simulink model "CruiseControl_V1"  (R2021b)
settings: Solver=FixedStepAuto  StartTime=0.0  StopTime=30  FixedStep=Ts  RelTol=1e-3
undefined symbols (not defined in the file): A, Cd, Crr, DiscIntNeverNeededParam, FaultInjection, FbrakeMax, Fmax, g, Kaw, ki, kp, Mass, rho, Ts, V0
settings Model: SimulationMode=software-in-the-loop (sil)  SILPILSimulationModeModelRef=accelerator  Creator=QNH2KOR  LastModifiedBy=QNH2KOR
settings OptimizationCC: DefaultParameterBehavior=Inlined  EnhancedBackFolding=on  PassReuseOutputArgsAs=Individual arguments  ZeroExternalMemoryAtStartup=off  ZeroInternalMemoryAtStartup=off  OptimizeBlockOrder=speed  DifferentSizesBufferReuse=on  OptimizationCustomize=off  EfficientTunableParamExpr=on
settings DebuggingCC: ParameterTunabilityLossMsg=error
settings SFSimCC: MATLABDynamicMemAlloc=off
settings RTWCC: Description=Embedded Coder  SystemTargetFile=ert.tlc  GenCodeOnly=on  TemplateMakefile=ert_default_tmf
settings CodeAppCC: ForceParamTrailComments=on  IgnoreCustomStorageClasses=off  OperatorAnnotations=on  SimulinkDataObjDesc=on  SFDataObjDesc=on  InsertBlockDesc=on
settings ERTTargetCC: TargetLangStandard=C99 (ISO)  GenerateSampleERTMain=on  SupportContinuousTime=on  InlinedParameterPlacement=NonHierarchical  ERTCustomFileTemplate=example_file_process.tlc

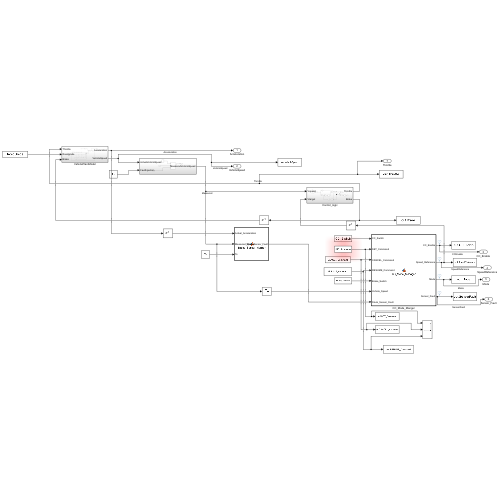
[thumbnail: Simulink's stored preview of the top-level diagram]
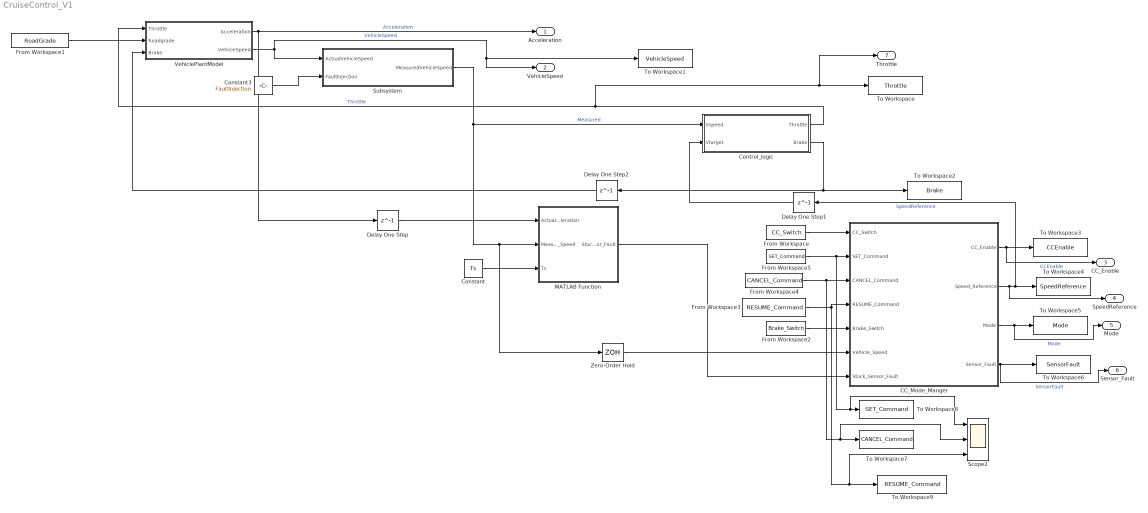
== system CruiseControl_V1 ==
  CC_Mode_Manger : MATLAB Function  TreatAsAtomicUnit=on
  Constant : Constant  Value=Ts
  Constant3 : Constant  Value=FaultInjection  SampleTime=Ts
  Control_logic : Subsystem
  Delay One Step : Delay  DelayLength=1  SampleTime=Ts
  Delay One Step1 : Delay  DelayLength=1  SampleTime=Ts
  Delay One Step2 : Delay  DelayLength=1  SampleTime=Ts
  From Workspace : FromWorkspace  VariableName=CC_Switch  SampleTime=Ts
  From Workspace1 : FromWorkspace  VariableName=RoadGrade  SampleTime=Ts  Interpolate=off  OutputAfterFinalValue=Holding final value
  From Workspace2 : FromWorkspace  VariableName=Brake_Switch  SampleTime=Ts
  From Workspace3 : FromWorkspace  VariableName=RESUME_Command  SampleTime=-1  Interpolate=off  OutputAfterFinalValue=Setting to zero
  From Workspace4 : FromWorkspace  VariableName=CANCEL_Command  SampleTime=Ts  Interpolate=off  OutputAfterFinalValue=Setting to zero
  From Workspace5 : FromWorkspace  VariableName=SET_Command  SampleTime=Ts  Interpolate=off  OutputAfterFinalValue=Setting to zero
  MATLAB Function : MATLAB Function  TreatAsAtomicUnit=on
  Scope2 : Scope  NumInputPorts=3
  Subsystem : Subsystem
  To Workspace : ToWorkspace  VariableName=Throttle  SaveFormat=Timeseries  SampleTime=-1
  To Workspace1 : ToWorkspace  VariableName=VehicleSpeed  SaveFormat=Timeseries  SampleTime=-1
  To Workspace2 : ToWorkspace  VariableName=Brake  SaveFormat=Timeseries  SampleTime=-1
  To Workspace3 : ToWorkspace  VariableName=CCEnable  SaveFormat=Timeseries  SampleTime=-1
  To Workspace4 : ToWorkspace  VariableName=SpeedReference  SaveFormat=Timeseries  SampleTime=-1
  To Workspace5 : ToWorkspace  VariableName=Mode  SaveFormat=Timeseries  SampleTime=-1
  To Workspace6 : ToWorkspace  VariableName=SensorFault  SaveFormat=Timeseries  SampleTime=-1
  To Workspace7 : ToWorkspace  VariableName=CANCEL_Command  SaveFormat=Timeseries  SampleTime=-1
  To Workspace8 : ToWorkspace  VariableName=SET_Command  SaveFormat=Timeseries  SampleTime=-1
  To Workspace9 : ToWorkspace  VariableName=RESUME_Command  SaveFormat=Timeseries  SampleTime=-1
  VehiclePlantModel : Subsystem
  Zero-Order Hold : ZeroOrderHold  SampleTime=-1
  Acceleration : Outport
  VehicleSpeed : Outport  Port=2
  CC_Enable : Outport  Port=3
  SpeedReference : Outport  Port=4
  Mode : Outport  Port=5
  Sensor_Fault : Outport  Port=6
  Throttle : Outport  Port=7
  wires:
  Control_logic/1(Throttle) -> Throttle/1, To Workspace/1, VehiclePlantModel/1(Throttle)  "Throttle"
  From Workspace1/1 -> VehiclePlantModel/2(Roadgrade)
  VehiclePlantModel/1(Acceleration) -> Acceleration/1, Delay One Step/1  "Acceleration"
  CC_Mode_Manger/1(CC_Enable) -> CC_Enable/1, To Workspace3/1  "CCEnable"
  Control_logic/2(Brake) -> Delay One Step2/1, To Workspace2/1
  VehiclePlantModel/2(VehicleSpeed) -> Subsystem/1(ActualVehicleSpeed), VehicleSpeed/1, To Workspace1/1  "VehicleSpeed"
  Constant3/1 -> Subsystem/2(FaultInjection)
  Constant/1 -> MATLAB Function/3(Ts)
  MATLAB Function/1(Stuck_Sensor_Fault) -> CC_Mode_Manger/7(Stuck_Sensor_Fault)
  From Workspace/1 -> CC_Mode_Manger/1(CC_Switch)
  From Workspace5/1 -> Scope2/1, To Workspace8/1, CC_Mode_Manger/2(SET_Command)
  From Workspace4/1 -> Scope2/2, To Workspace7/1, CC_Mode_Manger/3(CANCEL_Command)
  From Workspace3/1 -> CC_Mode_Manger/4(RESUME_Command), Scope2/3, To Workspace9/1
  From Workspace2/1 -> CC_Mode_Manger/5(Brake_Switch)
  CC_Mode_Manger/3(Mode) -> Mode/1, To Workspace5/1  "Mode"
  CC_Mode_Manger/2(Speed_Reference) -> SpeedReference/1, Delay One Step1/1, To Workspace4/1  "SpeedReference"
  Subsystem/1(MeasuredVehicleSpeed) -> Zero-Order Hold/1, MATLAB Function/2(Measured_Speed), Control_logic/1(Vspeed)  "Measured"
  Delay One Step/1 -> MATLAB Function/1(Actual_Acceleration)
  Delay One Step2/1 -> VehiclePlantModel/3(Brake)
  Delay One Step1/1 -> Control_logic/2(Vtarget)
  Zero-Order Hold/1 -> CC_Mode_Manger/6(Vehicle_Speed)
  CC_Mode_Manger/4(Sensor_Fault) -> Sensor_Fault/1, To Workspace6/1  "SensorFault"

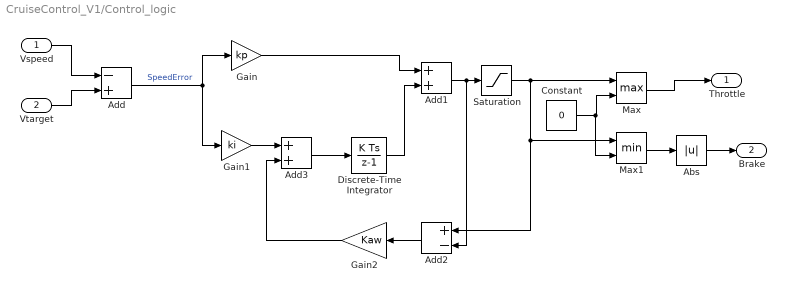
== system CruiseControl_V1/Control_logic ==
  Vspeed : Inport
  Vtarget : Inport  Port=2
  Abs : Abs
  Add : Sum  Inputs=-+
  Add1 : Sum
  Add2 : Sum  Inputs=+-
  Add3 : Sum
  Constant : Constant  Value=0
  Discrete-Time Integrator : DiscreteIntegrator  SampleTime=Ts  ICPrevOutput=DiscIntNeverNeededParam  ICPrevScaledInput=DiscIntNeverNeededParam
  Gain : Gain  Gain=kp
  Gain1 : Gain  Gain=ki
  Gain2 : Gain  Gain=Kaw
  Max : MinMax  Function=max  Inputs=2
  Max1 : MinMax  Inputs=2
  Saturation : Saturate  UpperLimit=1  LowerLimit=-1
  Throttle : Outport
  Brake : Outport  Port=2
  wires:
  Vtarget/1 -> Add/2
  Vspeed/1 -> Add/1
  Add/1 -> Gain1/1, Gain/1  "SpeedError"
  Gain/1 -> Add1/1
  Add1/1 -> Add2/2, Saturation/1
  Add2/1 -> Gain2/1
  Gain1/1 -> Add3/1
  Gain2/1 -> Add3/2
  Max/1 -> Throttle/1
  Constant/1 -> Max1/2, Max/2
  Saturation/1 -> Max/1, Max1/1, Add2/1
  Max1/1 -> Abs/1
  Abs/1 -> Brake/1
  Add3/1 -> Discrete-Time Integrator/1
  Discrete-Time Integrator/1 -> Add1/2

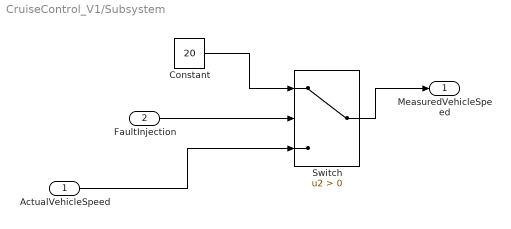
== system CruiseControl_V1/Subsystem ==
  ActualVehicleSpeed : Inport
  FaultInjection : Inport  Port=2
  Constant : Constant  Value=20
  Switch : Switch  Criteria=u2 > Threshold
  MeasuredVehicleSpeed : Outport
  wires:
  Switch/1 -> MeasuredVehicleSpeed/1
  ActualVehicleSpeed/1 -> Switch/3
  FaultInjection/1 -> Switch/2
  Constant/1 -> Switch/1

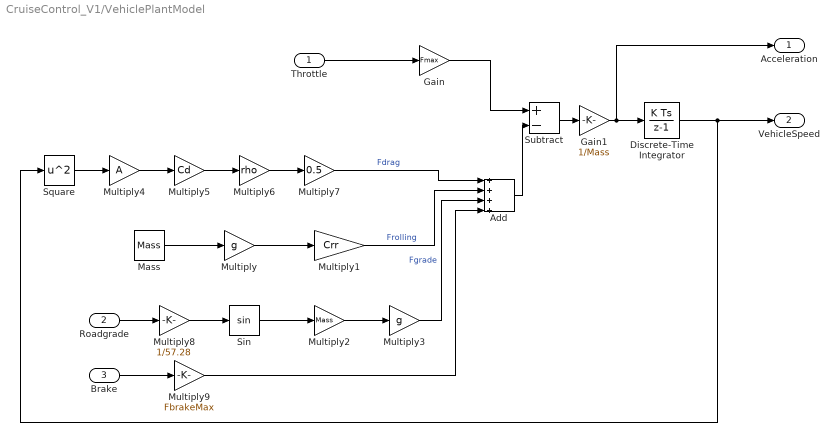
== system CruiseControl_V1/VehiclePlantModel ==
  Throttle : Inport
  Roadgrade : Inport  Port=2
  Brake : Inport  Port=3
  Add : Sum  Inputs=++++
  Discrete-Time Integrator : DiscreteIntegrator  InitialCondition=V0  SampleTime=Ts  ICPrevOutput=DiscIntNeverNeededParam  ICPrevScaledInput=DiscIntNeverNeededParam
  Gain : Gain  Gain=Fmax
  Gain1 : Gain  Gain=1/Mass
  Mass : Constant  Value=Mass
  Multiply : Gain  Gain=g
  Multiply1 : Gain  Gain=Crr
  Multiply2 : Gain  Gain=Mass
  Multiply3 : Gain  Gain=g
  Multiply4 : Gain  Gain=A
  Multiply5 : Gain  Gain=Cd
  Multiply6 : Gain  Gain=rho
  Multiply7 : Gain  Gain=0.5
  Multiply8 : Gain  Gain=1/57.28
  Multiply9 : Gain  Gain=FbrakeMax
  Sin : Trigonometry
  Square : Math  Operator=square  SaturateOnIntegerOverflow=on
  Subtract : Sum  Inputs=+-
  Acceleration : Outport
  VehicleSpeed : Outport  Port=2
  wires:
  Multiply7/1 -> Add/1  "Fdrag"
  Gain/1 -> Subtract/1
  Subtract/1 -> Gain1/1
  Square/1 -> Multiply4/1
  Multiply1/1 -> Add/2  "Frolling"
  Multiply3/1 -> Add/3  "Fgrade"
  Multiply5/1 -> Multiply6/1
  Multiply4/1 -> Multiply5/1
  Multiply6/1 -> Multiply7/1
  Multiply/1 -> Multiply1/1
  Multiply2/1 -> Multiply3/1
  Mass/1 -> Multiply/1
  Throttle/1 -> Gain/1
  Add/1 -> Subtract/2
  Gain1/1 -> Discrete-Time Integrator/1, Acceleration/1
  Discrete-Time Integrator/1 -> Square/1, VehicleSpeed/1
  Roadgrade/1 -> Multiply8/1
  Sin/1 -> Multiply2/1
  Multiply8/1 -> Sin/1
  Brake/1 -> Multiply9/1
  Multiply9/1 -> Add/4

== matlab function CruiseControl_V1/MATLAB Function ==
  settings: updateMethod=DISCRETE
  data: Actual_Acceleration input; Stuck_Sensor_Fault output; Measured_Speed input; Ts input

function Stuck_Sensor_Fault = Speed_Sensor_Monitor( ...
    Actual_Acceleration, Measured_Speed, Ts)

persistent elapsed_time
persistent initial_speed
persistent expected_speed_change
persistent fault_detected

if isempty(elapsed_time)
    elapsed_time = 0;
    initial_speed = Measured_Speed;
    expected_speed_change = 0;
    fault_detected = false;
end

% Accumulate expected speed change from actual acceleration
expected_speed_change = expected_speed_change + ...
                        Actual_Acceleration * Ts;

elapsed_time = elapsed_time + Ts;

% Evaluate once every 2 seconds
if elapsed_time >= 2.0

    measured_speed_change = Measured_Speed - initial_speed;

    % Detect significant expected change but negligible
    % measured speed change
    if abs(expected_speed_change) > 1.0 && ...
       abs(measured_speed_change) < 0.05

        fault_detected = true;
    end

    % Start next monitoring window
    elapsed_time = 0;
    initial_speed = Measured_Speed;
    expected_speed_change = 0;
end

% Fault remains latched until simulation restart
Stuck_Sensor_Fault = fault_detected;

end

== matlab function CruiseControl_V1/CC_Mode_Manger ==
  data: CC_Switch input; CC_Enable output; SET_Command input; CANCEL_Command input; RESUME_Command input; Brake_Switch input; Vehicle_Speed input; Speed_Reference output; Mode output; Sensor_Fault output; Stuck_Sensor_Fault input
 
function [CC_Enable, Speed_Reference, Mode,Sensor_Fault] = ...
    CC_Mode_Manager(CC_Switch, SET_Command, ...
    CANCEL_Command, RESUME_Command, ...
    Brake_Switch, Vehicle_Speed,Stuck_Sensor_Fault)

persistent state stored_speed

Sensor_Fault = isnan(Vehicle_Speed) || ...
               isinf(Vehicle_Speed) || ...
               Vehicle_Speed < 0 || ...
               Vehicle_Speed > 60 || ...
               Stuck_Sensor_Fault;
 
if isempty(state)
    state = 0;          % OFF
    stored_speed = 0;
end

% Master cruise-control switch
if ~CC_Switch
    state = 0;
    stored_speed = 0;

elseif Sensor_Fault
    state = 1;

else
    switch state

        case 0  % OFF
            state = 1;  % STANDBY

        case 1  % STANDBY

            if Brake_Switch
                    state = 1;

            elseif SET_Command && Vehicle_Speed > 0
                stored_speed = Vehicle_Speed;
                state = 2;

            elseif RESUME_Command && stored_speed > 0
                state = 2;
            end

        case 2  % ACTIVE

            if CANCEL_Command || Brake_Switch
                stored_speed = Vehicle_Speed;
                state = 1;
            end

    end
end

% Outputs
CC_Enable = (state == 2);
Speed_Reference = stored_speed;
Mode = state;

end
